simulink model "ME598A_Final_Project_R6"  (R2025b)
settings: Solver=ode23t  StartTime=0.0  StopTime=inf  RelTol=1e-3
InitFcn:
  | RPInit
model workspace (MAT data in the model file):
  mapForSim.obsMap = [0 0 0 0 0 0 0 0 0 0 0 0 ... (4194304 elements, 2048x2048)]
  mapForSim.scaleFactor = 409.6
  mapForSim.simMap = robotics.BinaryOccupancyGrid
  mapForSim.simMap.Grid = [1 1 1 1 1 1 1 1 1 1 1 1 ... (4194304 elements, 2048x2048)]
  mapForSim.simMap.SharedProperties = matlabshared.autonomous.internal.SharedMapProperties
  mapForSim.simMap.SharedProperties.Resolution = 409.6
  mapForSim.simMap.SharedProperties.GridSize = [2048 2048]
  mapForSim.simMap.SharedProperties.XLocalLimits = [0 5]
  mapForSim.simMap.SharedProperties.YLocalLimits = [0 5]
  mapForSim.simMap.SharedProperties.XWorldLimits = [0 5]
  mapForSim.simMap.SharedProperties.YWorldLimits = [0 5]
  mapForSim.simMap.SharedProperties.Width = 5
  mapForSim.simMap.SharedProperties.Height = 5
  mapForSim.simMap.SharedProperties.LocalOriginInWorldInternal = [0 0]
  mapForSim.simMap.LayerName = 'binaryLayer'
  mapForSim.simMap.DataType = 'logical'
  mapForSim.simMap.Buffer = matlabshared.autonomous.internal.CircularBuffer
  mapForSim.simMap.Buffer.ConstVal = 0
  mapForSim.simMap.Buffer.DataType = 'logical'
  mapForSim.simMap.Buffer.Index = matlabshared.autonomous.internal.CircularBufferIndex
  mapForSim.simMap.Buffer.Index.Head = [1 1]
  mapForSim.simMap.Buffer.Index.Size = [2048 2048]
  mapForSim.simMap.Buffer.Index.NewRegions = [0 0 0 0]
  mapForSim.simMap.Buffer.Index.DropEntireMap = 0
  mapForSim.simMap.Buffer.Index.DropTwoRegions = [0 0]
  mapForSim.simMap.Buffer.Buffer = [1 1 1 1 1 1 1 1 1 1 1 1 ... (4194304 elements, 2048x2048)]
  mapForSim.simMap.Buffer.BufferSize = [2048 2048 1]
  mapForSim.simMap.DefaultValueInternal = 0
  mapForSim.simMap.DataSize = [2048 2048]
  occGrid = robotics.BinaryOccupancyGrid
  occGrid.Grid = [1 1 1 1 1 1 1 1 1 1 1 1 ... (4194304 elements, 2048x2048)]
  occGrid.SharedProperties = matlabshared.autonomous.internal.SharedMapProperties
  occGrid.SharedProperties.Resolution = 409.6
  occGrid.SharedProperties.GridSize = [2048 2048]
  occGrid.SharedProperties.XLocalLimits = [0 5]
  occGrid.SharedProperties.YLocalLimits = [0 5]
  occGrid.SharedProperties.XWorldLimits = [0 5]
  occGrid.SharedProperties.YWorldLimits = [0 5]
  occGrid.SharedProperties.Width = 5
  occGrid.SharedProperties.Height = 5
  occGrid.SharedProperties.LocalOriginInWorldInternal = [0 0]
  occGrid.LayerName = 'binaryLayer'
  occGrid.DataType = 'logical'
  occGrid.Buffer = matlabshared.autonomous.internal.CircularBuffer
  occGrid.Buffer.ConstVal = 0
  occGrid.Buffer.DataType = 'logical'
  occGrid.Buffer.Index = matlabshared.autonomous.internal.CircularBufferIndex
  occGrid.Buffer.Index.Head = [1 1]
  occGrid.Buffer.Index.Size = [2048 2048]
  occGrid.Buffer.Index.NewRegions = [0 0 0 0]
  occGrid.Buffer.Index.DropEntireMap = 0
  occGrid.Buffer.Index.DropTwoRegions = [0 0]
  occGrid.Buffer.Buffer = [1 1 1 1 1 1 1 1 1 1 1 1 ... (4194304 elements, 2048x2048)]
  occGrid.Buffer.BufferSize = [2048 2048 1]
  occGrid.DefaultValueInternal = 0
  occGrid.DataSize = [2048 2048]
undefined symbols (not defined in the file): Base, FloorSurface, PlowSurface, Ref, RobotSurface, Side1, Side2, X, Y, Z
libraries: sm_lib x27, nesl_utility x11, RP_Simulator_Components x7, ME598_ProjectLibrary x3, RoboticsPlayground x2
(part 1 of 2)
settings Model: PacingRate=1000  Creator=josea  LastModifiedBy=beaut
settings SolverCC: AlgebraicLoopSolver=TrustRegion
settings DataIOCC: ReturnWorkspaceOutputs=off
settings DebuggingCC: UnconnectedInputMsg=warning  UnconnectedOutputMsg=warning  ArithmeticOperatorsInVariantConditions=warning
settings ModelReferenceCC: EnableRefExpFcnMdlSchedulingChecks=on
settings SFSimCC: SimUseLocalCustomCode=off  CustomCodeUndefinedFunction=UseInterfaceOnly
settings RTWCC: RTWUseLocalCustomCode=off  GPUComputeCapability=3.5  DLArmComputeVersion=19.05
settings DiagnosticsConfigSet: SimMechanicsRigidlyBoundBlock=none
settings ExplorerConfigSet: InternalSimMechanicsExplorerSettings="<ExplorerConfiguration><canonicalview>default</canonicalview><TilePanel><TileInfo><Tiles Columns=\"2\" Count=\"3\" Height=\"704\" Rows=\"2\" Width=\"1079\"><Row Weight=\"0.4995\"/><Row Weight=\"0.5005\"/><Column Weight=\"0.4996\"/><Column Weight=\"0.5004\"/><Tile Height=\"1\" Width=\"2\" X=\"0\" Y=\"0\"/><Tile Height=\"1\" Width=\"1\" X=\"0\" Y=\"1\"/><Tile Height=\"1\" Width=\"1\" X=\"1\" Y=\"1\"/></Tiles></TileInfo><SceneInfo><SceneViewer><IsThisViewStd><IsStandardView>off</IsStandardView><StandardViewName>Front</StandardViewName></IsThisViewStd><BGColor><R>0.60000002384185791</R><G>0.60000002384185791</G><B>0.60000002384185791</B><A>1</A></BGColor><Camera><DoPerspective>off</DoPerspective><Position><X>-0.86116534267326283</X><Y>0.23588412890430099</Y><Z>21.59798</Z></Position><Center><X>-0.86116534267326283</X><Y>0.23588412890430099</Y><Z>0.12587000000000001</Z></Center><Up><X>0</X><Y>1</Y><Z>0</Z></Up><XLim>3.0477928446452562</XLim><YLim>3.0477928446452562</YLim><ViewLimDist>0.01</ViewLimDist></Camera></SceneViewer><SceneViewer><IsThisViewStd><IsStandardView>off</IsStandardView><StandardViewName>Front</StandardViewName></IsThisViewStd><BGColor><R>0.60000002384185791</R><G>0.60000002384185791</G><B>0.60000002384185791</B><A>1</A></BGColor><Camera><DoPerspective>on</DoPerspective><Position><X>-0.46788000000000002</X><Y>0.21970000000000001</Y><Z>0.45108999999999999</Z></Position><Center><X>0.46222000000000002</X><Y>0.085760000000000003</Y><Z>0.10907</Z></Center><Up><X>0.33852730030170697</X><Y>-0.048749611226549958</Y><Z>0.9396928978957424</Z></Up><XLim>0.46630765815499858</XLim><YLim>0.46630765815499858</YLim><ViewLimDist>0.01</ViewLimDist></Camera></SceneViewer><SceneViewer><IsThisViewStd><IsStandardView>off</IsStandardView><StandardViewName>Front</StandardViewName></IsThisViewStd><BGColor><R>0.60000002384185791</R><G>0.60000002384185791</G><B>0.60000002384185791</B><A>1</A></BGColor><Camera><DoPerspective>off</DoPerspective><Position><X>0</X><Y>0</Y><Z>21.59798</Z></Position><Center><X>0</X><Y>0</Y><Z>0.12587000000000001</Z></Center><Up><X>0</X><Y>1</Y><Z>0</Z></Up><XLim>2.5955999995395542</XLim><YLim>2.5955999995395542</YLim><ViewLimDist>0.01</ViewLimDist></Camera></SceneViewer></SceneInfo></TilePanel><MechEditorPanel><GfxPanelCameraMap><MapElement CameraMLId=\"Camera1\" GfxPanelIndex=\"1\"/></GfxPanelCameraMap><Cameras><Camera><Id>Camera1</Id><Value><Name>RobotView</Name><NativeCamera><PositionTrackingFeature>Object_Environment_ME_598.Plow_Tank_Robot.Body.RobotCamera.F</PositionTrackingFeature><CenterTrackingFeature>Object_Environment_ME_598.Plow_Tank_Robot.Body.RobotCamera.F</CenterTrackingFeature><UpVectorTrackingFeature>Object_Environment_ME_598.Plow_Tank_Robot.Body.RobotCamera.F</UpVectorTrackingFeature><CenterTrackingOrigin>off</CenterTrackingOrigin><CenterTrackingDirection>+X</CenterTrackingDirection><UpVectorTrackingDirection>+Z</UpVectorTrackingDirection></NativeCamera></Value></Camera></Cameras><VideoCreator><IncludeTiles>Selected</IncludeTiles><IncludeTime>on</IncludeTime><IncludeWorldFrame>off</IncludeWorldFrame><PlaybackSpeedRatio>1</PlaybackSpeedRatio><FrameRate>30</FrameRate><FrameSize>auto</FrameSize><VideoFormat>MotionJPEGAVI</VideoFormat></VideoCreator></MechEditorPanel><PlaybackSettings><PlaybackSpeedFactor>4</PlaybackSpeedFactor></PlaybackSettings></ExplorerConfiguration>"

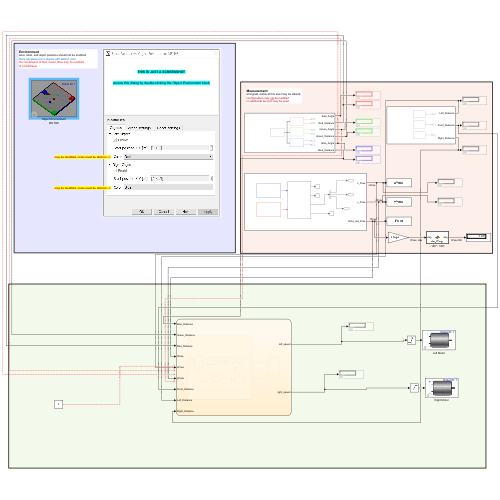
[thumbnail: Simulink's stored preview of the top-level diagram]
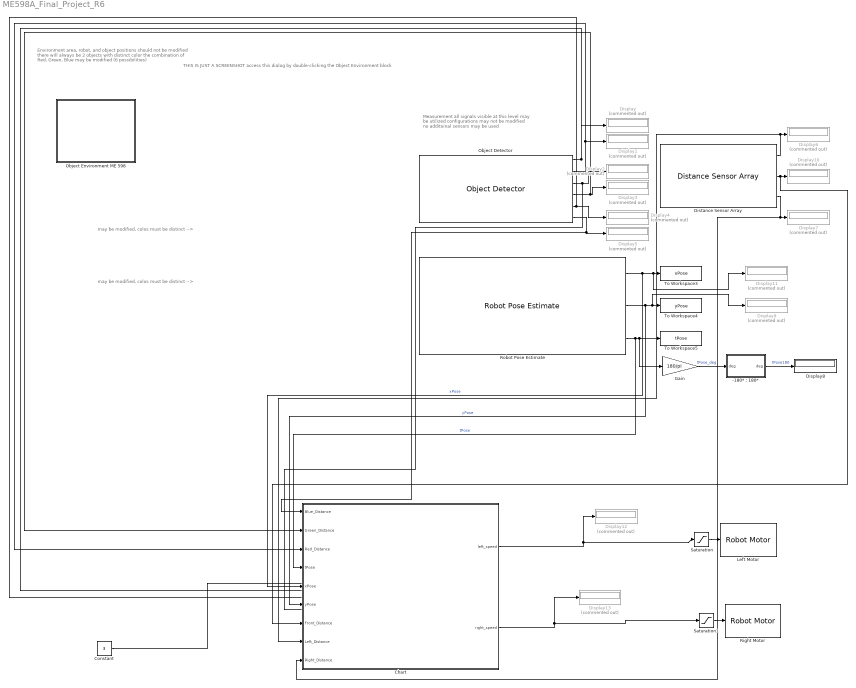
== system ME598A_Final_Project_R6 ==
  note: Environment
      | area, robot, and object positions should not be modified
      | there will always be 2 objects with distinct color
      | the combination of Red, Green, Blue may be modified
      | (6 possibilities)
  note: Measurement
      | all signals visible at this level may be utilized configurations may not be modified
      | no additoinal sensors may be used
  note: may be modified, colos must be distinct -->
  note: THIS IS JUST A SCREENSHOT
      |
      | access this dialog by double-clicking the Object Environment block
  note: may be modified, colos must be distinct -->
  "-180* : 180*" : MATLAB Function  TreatAsAtomicUnit=on
  Chart : Stateflow chart  TreatAsAtomicUnit=on
  Constant : Constant  Value=3
  Display{,1..7,9..13} (13 alike) : Display  Commented=on
  Display8 : Display
  Distance Sensor Array : ME598_ProjectLibrary/Distance Sensor Array
  Gain : Gain  Gain=180/pi
  Left Motor : RoboticsPlayground/Basic Sensors and Actuators/Robot Motor  robotId=1  motorChoice=1
      settings: SourceProductName=Robotics Playground
  Object Detector : ME598_ProjectLibrary/Object Detector
  Object Environment ME 598 : Subsystem  mask(RP Object Environment){obj1=on, objPose1=[0 1.5], objColor1=Green, obj2=off, objPose2=[0 0], objColor2=Green, obj3=on, objPose3=[0 -1.5], objColor3=Red, obj4=off, objPose4=[-0.61298      2.9263], objColor4=Red, obj5=off, objPose5=[-0.61298      2.9263], objColor5=Red, arenaLength=5, arenaWidth=5, robotId=1, wheelBase=0.5, wheelRadius=0.1, robotColor=[0.5 0 0], startPose=[-1.5 -1.5]}
      mask prompts: obj1 "Enabled"; objPose1 "Initial position X Y [m]"; objColor1 "Color"; obj2 "Enabled"; objPose2 "Initial position X Y [m]"; objColor2 "Color"; obj3 "Enabled"; objPose3 "Initial position X Y [m]"; objColor3 "Color"; obj4 "Enabled"; objPose4 "Initial position X Y [m]"; objColor4 "Color"; obj5 "Enabled"; objPose5 "Initial position X Y [m]"; objColor5 "Color"; arenaLength "Length [m]"; arenaWidth "Width [m]"; robotId "Robot ID"; wheelBase "Distance between wheels [m]"; wheelRadius "Wheel radius [m]"; robotColor "Color [R G B]"; startPose "Initial Position X Y [m]"
      mask help:
      | This block has been customized and tested with MATLAB R2025b and Robotics Playground v23.1.1.0
      | for Stevens Institute of Technology course ME 598, Spring 2026.
      |
      | It contains a virtual environment for a single robot to interact with walls and moveable objects. For your course project, only the sensors and actuators provided in the file ** Project_start.slx ** may be used for sensing and to actuate the robot.
      |
      | Motor mapping for the robot is as follows:
      |
      | Motor 1 -> Left wheel motor **torque**
      | Motor 2 -> Right wheel motor **torque**
      settings: CopyFcn=|
      | set_param(gcs,'InitFcn','RPInit');
      | set_param(gcs,'Solver','ode23t');
      | set_param(gcs, 'EnablePacing', 'on')
      | set_param(gcs, 'PacingRate', 1)
      mask Help: web('object_arena.htm')
      mask Callback obj1: setObjects(gcb)
      mask Callback objPose1: setObjects(gcb)
      mask TypeOptions objColor1: Red | Green | Blue
      mask Callback objColor1: setObjects(gcb)
      mask Callback obj2: setObjects(gcb)
      mask Callback objPose2: setObjects(gcb)
      mask TypeOptions objColor2: Red | Green | Blue
      mask Callback objColor2: setObjects(gcb)
      mask Callback obj3: setObjects(gcb)
      mask Callback objPose3: setObjects(gcb)
      mask TypeOptions objColor3: Red | Green | Blue
      mask Callback objColor3: setObjects(gcb)
      mask Callback obj4: setObjects(gcb)
      mask Callback objPose4: setObjects(gcb)
      mask TypeOptions objColor4: Red | Green | Blue
      mask Callback objColor4: setObjects(gcb)
      mask Callback obj5: setObjects(gcb)
      mask Callback objPose5: setObjects(gcb)
      mask TypeOptions objColor5: Red | Green | Blue
      mask Callback objColor5: setObjects(gcb)
      mask DialogControl objT Prompt: Object settings
      mask DialogControl objc1 Prompt: Left Object
      mask DialogControl objc2 Prompt: Center Object
      mask DialogControl objc3 Prompt: Right Object
      mask DialogControl objc4 Prompt: Object 4
      mask DialogControl objc5 Prompt: Object 5
      mask DialogControl Container6 Prompt: Arena settings
      mask DialogControl Container4 Prompt: Robot settings
      mask Display:
      | color('white');
      | plot([100,100,100,100]*1,[100,100,100,100]*1);
      | plot([100,100,100,100]*0,[100,100,100,100]*0);
      | image('ObjectEnv.PNG')
      | color('blue');
      | id=eval(get_param(gcb,'robotId'));
      | text(99, 92, ['Robot ID: ' num2str(id)], 'horizontalAlignment', 'right');
  Right Motor : RoboticsPlayground/Basic Sensors and Actuators/Robot Motor  robotId=1  motorChoice=2
      settings: SourceProductName=Robotics Playground
  Robot Pose Estimate : ME598_ProjectLibrary/Robot Pose Estimate
  Saturation : Saturate  UpperLimit=127  LowerLimit=-127
  Saturation1 : Saturate  UpperLimit=127  LowerLimit=-127
  To Workspace3 : ToWorkspace  VariableName=xPose  SampleTime=-1
  To Workspace4 : ToWorkspace  VariableName=yPose  SampleTime=-1
  To Workspace5 : ToWorkspace  VariableName=tPose  SampleTime=-1
  wires:
  Object Detector/1 -> Display/1
  Object Detector/2 -> Chart/3(Red_Distance), Display1/1
  Object Detector/4 -> Chart/2(Green_Distance), Display3/1
  Object Detector/3 -> Display2/1
  Distance Sensor Array/1 -> Chart/8(Left_Distance), Display6/1
  Distance Sensor Array/3 -> Chart/9(Right_Distance), Display7/1
  Robot Pose Estimate/3 -> Chart/4(tPose), Gain/1, To Workspace5/1  "tPose"
  Gain/1 -> "-180* : 180*"/1("deg ")  "tPose_deg"
  Robot Pose Estimate/1 -> Chart/5(xPose), Display11/1, To Workspace3/1  "xPose"
  Robot Pose Estimate/2 -> Chart/6(yPose), Display9/1, To Workspace4/1  "yPose"
  Saturation/1 -> Left Motor/1
  Distance Sensor Array/2 -> Chart/7(Front_Distance), Display10/1
  "-180* : 180*"/1(deg) -> Display8/1  "tPose180"
  Object Detector/5 -> Display4/1
  Object Detector/6 -> Chart/1(Blue_Distance), Display5/1
  Saturation1/1 -> Right Motor/1
  Chart/1(left_speed) -> Display12/1, Saturation/1
  Chart/2(right_speed) -> Display13/1, Saturation1/1
  Constant/1 -> ?

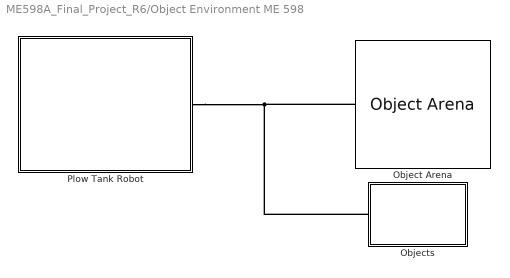
== system ME598A_Final_Project_R6/Object Environment ME 598 ==
  Object Arena : RP_Simulator_Components/Object Arena  length=arenaLength  width=arenaWidth  robotRadius=wheelBase/2
  Objects : Subsystem
  Plow Tank Robot : Subsystem  AncestorBlock=RoboticsPlayground/Environments/Object Environment/Plow Tank Robot  mask(RP Contact Tank Robot){robotId=robotId, wheelRadius=wheelRadius, wheelBase=wheelBase, wheelThickness=0.025, chassisThickness=0.05, startPose=startPose, choice=off, sensorTs=0.05, wheelMass=0.2, chassisMass=0.5, maxWheelTorque=1, floorSize=[arenaLength arenaWidth], wheelColor=[0.25 0.25 0.25], chassisColor=robotColor}
      mask prompts: robotId "Robot ID"; wheelRadius "Wheel Radius [m]"; wheelBase "Wheelbase [m]"; wheelThickness "Wheel Thickness [m]"; chassisThickness "Chassis Thickness [m]"; startPose "Start Position [m]"; choice "Reverse Start Position"; sensorTs "Sensor sample time [s]"; wheelMass "Wheel Mass [kg]"; chassisMass "Chassis Mass [kg]"; maxWheelTorque "Maximum wheel torque [N*m]"; floorSize "Floor Dimensions [m]"; wheelColor "Wheel Color"; chassisColor "Chassis Color"
      mask help:
      | This robot implements contact between the robot wheels and the floor of an arena. The stck-slip friction implemented using contact force libraries makes the robot behavior more realistic. The inputs to the robot are now motor torque, which is set using the Robotics Playground Motor blocks. The motor mappings are as follows:
      |
      | Motor 1 -> Left wheel motor torque
      | Motor 2 -> Right wheel motor torque
      mask init:
      | ID=num2str(eval(get_param(gcb,'robotId')));
      | block=gcb;
      | 
      | set_param([block '/motor1t'],'GotoTag',['R' ID 'motor1t']);
      | set_param([block '/motor2t'],'GotoTag',['R' ID 'motor2t']);
      | set_param([block '/motor1q'],'GotoTag',['R' ID 'motor1q']);
      | set_param([block '/motor1w'],'GotoTag',['R' ID 'motor1w']);
      | set_param([block '/motor2q'],'GotoTag',['R' ID 'motor2q']);
      | set_param([block '/motor2w'],'GotoTag',['R' ID 'motor2w']);
      | set_param([block '/xPose'],'GotoTag',['R' ID 'xPose']);
      | set_param([block '/yPose'],'GotoTag',['R' ID 'yPose']);
      | set_param([block '/tPose'],'GotoTag',['R' ID 'tPose']);
      | set_param([block '/tRate'],'GotoTag',['R' ID 'tRate']);
      | set_param([block '/tAngle'],'GotoTag',['R' ID 'tAngle']);
      | 
      | % Add sensor visuals
      | 
      | addSensors(block,eval(ID));
      mask DialogControl KinContainer Prompt: Kinematics
      mask DialogControl DynamicsContainer Prompt: Dynamics
      mask DialogControl AppearanceContainer Prompt: Appearance
      mask Display:
      | image('plowRobot.PNG')
      | port_label('Rconn',1,'RP-Bus')
  connections:
  Object Arena/LConn1 -- Plow Tank Robot/RConn1 -- Objects/LConn1

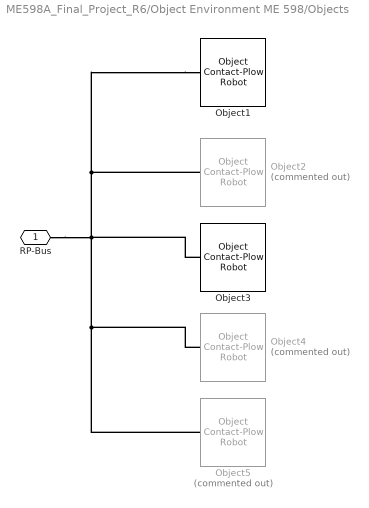
== system ME598A_Final_Project_R6/Object Environment ME 598/Objects ==
  Object1 : RP_Simulator_Components/Object Contact-Plow Robot  objectId=1  Pose=[0 1.5]  objRadius=0.15  robotRadius=0.25  height=0.2  color=[0 0.8 0]  length=arenaLength  width=arenaWidth
  Object2 : RP_Simulator_Components/Object Contact-Plow Robot  Commented=on  objectId=2  Pose=[0 0]  objRadius=0.15  robotRadius=0.25  height=0.2  color=[0 0.8 0]  length=arenaLength  width=arenaWidth
  Object3 : RP_Simulator_Components/Object Contact-Plow Robot  objectId=3  Pose=[0 -1.5]  objRadius=0.15  robotRadius=0.25  height=0.2  color=[0.8 0 0]  length=arenaLength  width=arenaWidth
  Object4 : RP_Simulator_Components/Object Contact-Plow Robot  Commented=on  objectId=4  Pose="[-0.61298      2.9263]"  objRadius=0.15  robotRadius=0.25  height=0.2  color=[0.8 0 0]  length=arenaLength  width=arenaWidth
  Object5 : RP_Simulator_Components/Object Contact-Plow Robot  Commented=on  objectId=5  Pose="[-0.61298      2.9263]"  objRadius=0.15  robotRadius=0.25  height=0.2  color=[0.8 0 0]  length=arenaLength  width=arenaWidth
  RP-Bus : PMIOPort  Side=Left
  connections:
  Object1/LConn1 -- Object3/LConn1 -- Object5/LConn1 -- Object4/LConn1 -- RP-Bus/RConn1 -- Object2/LConn1

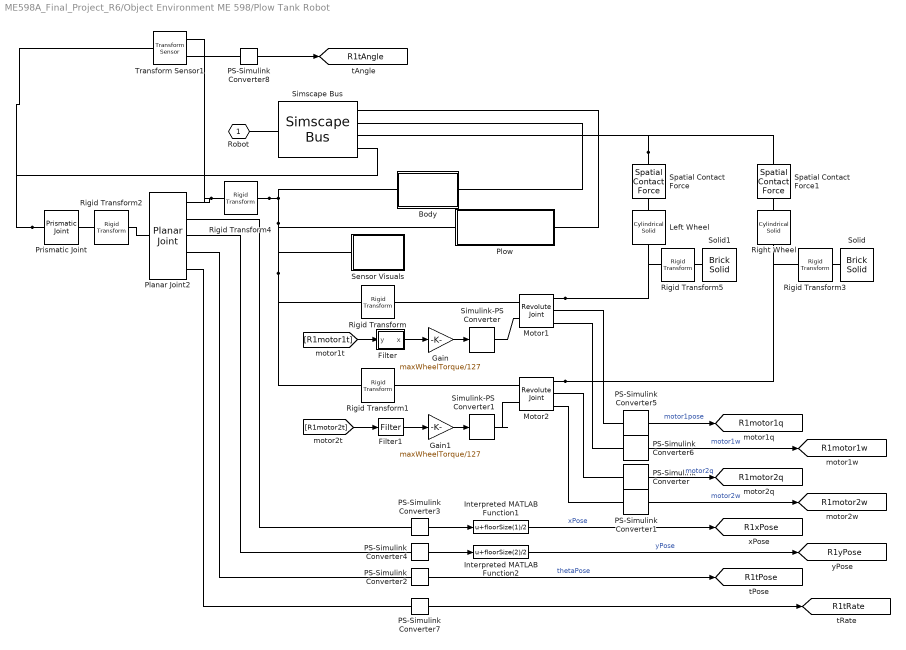
== system ME598A_Final_Project_R6/Object Environment ME 598/Plow Tank Robot ==
  Body : Subsystem
  Filter : Subsystem
  Filter1 : RP_Simulator_Components/Contact Tank Robot/Filter  SystemSampleTime=-1  VariantActivationTime=update diagram  EmptyChoice=off  PassThrough=off  PassThroughVariantControl=(default)  EmptyChoiceVariantControl=(default)  AllowFlexibleInterface=on  Latency=0  AutoFrameSizeCalculation=off
  Gain : Gain  Gain=maxWheelTorque/127
  Gain1 : Gain  Gain=maxWheelTorque/127
  Interpreted MATLAB Function1 : MATLABFcn  MATLABFcn=u+floorSize(1)/2
  Interpreted MATLAB Function2 : MATLABFcn  MATLABFcn=u+floorSize(2)/2
  Left Wheel : sm_lib/Body Elements/Cylindrical Solid  CylinderRadius=wheelRadius  CylinderRadiusUnits=m  CylinderLength=wheelThickness  CylinderLengthUnits=m  ExportEntireGeometry=on  InertiaType=CalculateFromGeometry  BasedOnType=Mass  Density=1000  DensityUnits=kg/m^3  Mass=wheelMass  MassUnits=kg  CenterOfMass=[0 0 0]  CenterOfMassUnits=m  MomentsOfInertia=[1 1 1]  MomentsOfInertiaUnits=kg*m^2  ProductsOfInertia=[1 1 1]  ProductsOfInertiaUnits=kg*m^2  GraphicType=FromGeometry  MarkerShape=Sphere  MarkerSize=10  GraphicVisPropType=SimpleVisualProperties  GraphicDiffuseColor=wheelColor  GraphicOpacity=1.0  GraphicSpecularColor=[0.5 0.5 0.5 1.0]  GraphicAmbientColor=[0.15 0.15 0.15 1.0]  GraphicEmissiveColor=[0.0 0.0 0.0 1.0]  GraphicShininess=75  DoExposeReferenceFrame=on  SerializedFrames=<Frames/>
  Motor1 : sm_lib/Joints/Revolute Joint  JointMode=Normal  CompositeWrenchDir=FollowerOnBase  CompositeWrenchFrame=BaseFrame  SenseConstraintForce=off  SenseConstraintTorque=off  SenseTotalForce=off  SenseTotalTorque=off  PositionTargetSpecify=off  PositionTargetPriority=High  PositionTargetValue=0  PositionTargetValueUnits=deg  VelocityTargetSpecify=off  VelocityTargetPriority=High  VelocityTargetValue=0  VelocityTargetValueUnits=deg/s  EquilibriumPosition=0  EquilibriumPositionUnits=deg  SpringStiffness=0  SpringStiffnessUnits=N*m/deg  DampingCoefficient=0.004  DampingCoefficientUnits=N*m/(deg/s)  LowerLimitSpecify=off  LowerLimitBound=-90  LowerLimitBoundUnits=deg  LowerLimitStiffness=1e4  LowerLimitStiffnessUnits=N*m/deg  LowerLimitDamping=10  LowerLimitDampingUnits=N*m/(deg/s)  LowerLimitTransitionRegionWidth=0.1  LowerLimitTransitionRegionWidthUnits=deg  UpperLimitSpecify=off  UpperLimitBound=90  UpperLimitBoundUnits=deg  UpperLimitStiffness=1e4  UpperLimitStiffnessUnits=N*m/deg  UpperLimitDamping=10  UpperLimitDampingUnits=N*m/(deg/s)  UpperLimitTransitionRegionWidth=0.1  UpperLimitTransitionRegionWidthUnits=deg  TorqueActuationMode=InputTorque  MotionActuationMode=ComputedMotion  SensePosition=on  SenseVelocity=on  SenseAcceleration=off  SenseTorqueForce=off  SenseLowerLimitTorqueForce=off  SenseUpperLimitTorqueForce=off
  Motor2 : sm_lib/Joints/Revolute Joint  JointMode=Normal  CompositeWrenchDir=FollowerOnBase  CompositeWrenchFrame=BaseFrame  SenseConstraintForce=off  SenseConstraintTorque=off  SenseTotalForce=off  SenseTotalTorque=off  PositionTargetSpecify=off  PositionTargetPriority=High  PositionTargetValue=0  PositionTargetValueUnits=deg  VelocityTargetSpecify=off  VelocityTargetPriority=High  VelocityTargetValue=0  VelocityTargetValueUnits=deg/s  EquilibriumPosition=0  EquilibriumPositionUnits=deg  SpringStiffness=0  SpringStiffnessUnits=N*m/deg  DampingCoefficient=0.004  DampingCoefficientUnits=N*m/(deg/s)  LowerLimitSpecify=off  LowerLimitBound=-90  LowerLimitBoundUnits=deg  LowerLimitStiffness=1e4  LowerLimitStiffnessUnits=N*m/deg  LowerLimitDamping=10  LowerLimitDampingUnits=N*m/(deg/s)  LowerLimitTransitionRegionWidth=0.1  LowerLimitTransitionRegionWidthUnits=deg  UpperLimitSpecify=off  UpperLimitBound=90  UpperLimitBoundUnits=deg  UpperLimitStiffness=1e4  UpperLimitStiffnessUnits=N*m/deg  UpperLimitDamping=10  UpperLimitDampingUnits=N*m/(deg/s)  UpperLimitTransitionRegionWidth=0.1  UpperLimitTransitionRegionWidthUnits=deg  TorqueActuationMode=InputTorque  MotionActuationMode=ComputedMotion  SensePosition=on  SenseVelocity=on  SenseAcceleration=off  SenseTorqueForce=off  SenseLowerLimitTorqueForce=off  SenseUpperLimitTorqueForce=off
  PS-Simulink Converter{,1,3..6} (6 alike) : nesl_utility/PS-Simulink Converter  PhysicalDomain=network_engine_domain  SubClassName=ps_output  LeftPortType=input  RightPortType=output  PseudoPeriodic=off  Frequencies=[]  VectorFormat=1-D array  Unit=1  AffineConversion=off
  PS-Simulink Converter2 : nesl_utility/PS-Simulink Converter  PhysicalDomain=network_engine_domain  SubClassName=ps_output  LeftPortType=input  RightPortType=output  PseudoPeriodic=off  Frequencies=[]  VectorFormat=1-D array  Unit=rad  AffineConversion=off
  PS-Simulink Converter7 : nesl_utility/PS-Simulink Converter  PhysicalDomain=network_engine_domain  SubClassName=ps_output  LeftPortType=input  RightPortType=output  PseudoPeriodic=off  Frequencies=[]  VectorFormat=1-D array  Unit=deg/s  AffineConversion=off
  PS-Simulink Converter8 : nesl_utility/PS-Simulink Converter  PhysicalDomain=network_engine_domain  SubClassName=ps_output  LeftPortType=input  RightPortType=output  PseudoPeriodic=off  Frequencies=[]  VectorFormat=1-D array  Unit=deg  AffineConversion=off
  Planar Joint2 : sm_lib/Joints/Planar Joint  JointMode=Normal  CompositeWrenchDir=FollowerOnBase  CompositeWrenchFrame=BaseFrame  SenseConstraintForce=off  SenseConstraintTorque=off  SenseTotalForce=off  SenseTotalTorque=off  PxPositionTargetSpecify=on  PxPositionTargetPriority=High  PxPositionTargetValue=startPose(1)  PxPositionTargetValueUnits=m  PxVelocityTargetSpecify=off  PxVelocityTargetPriority=High  PxVelocityTargetValue=0  PxVelocityTargetValueUnits=m/s  PxEquilibriumPosition=0  PxEquilibriumPositionUnits=m  PxSpringStiffness=0  PxSpringStiffnessUnits=N/m  PxDampingCoefficient=5  PxDampingCoefficientUnits=N/(m/s)  PxLowerLimitSpecify=off  PxLowerLimitBound=-1  PxLowerLimitBoundUnits=m  PxLowerLimitStiffness=1e6  PxLowerLimitStiffnessUnits=N/m  PxLowerLimitDamping=1e3  PxLowerLimitDampingUnits=N/(m/s)  PxLowerLimitTransitionRegionWidth=1e-4  PxLowerLimitTransitionRegionWidthUnits=m  PxUpperLimitSpecify=off  PxUpperLimitBound=1  PxUpperLimitBoundUnits=m  PxUpperLimitStiffness=1e6  PxUpperLimitStiffnessUnits=N/m  PxUpperLimitDamping=1e3  PxUpperLimitDampingUnits=N/(m/s)  PxUpperLimitTransitionRegionWidth=1e-4  PxUpperLimitTransitionRegionWidthUnits=m  PxTorqueActuationMode=NoTorque  PxMotionActuationMode=ComputedMotion  PxSensePosition=on  PxSenseVelocity=off  PxSenseAcceleration=off  PxSenseTorqueForce=off  PxSenseLowerLimitTorqueForce=off  PxSenseUpperLimitTorqueForce=off  PyPositionTargetSpecify=on  PyPositionTargetPriority=High  PyPositionTargetValue=startPose(2)  PyPositionTargetValueUnits=m  PyVelocityTargetSpecify=off  PyVelocityTargetPriority=High  PyVelocityTargetValue=0  PyVelocityTargetValueUnits=m/s  PyEquilibriumPosition=0  PyEquilibriumPositionUnits=m  PySpringStiffness=0  PySpringStiffnessUnits=N/m  PyDampingCoefficient=5  PyDampingCoefficientUnits=N/(m/s)  PyLowerLimitSpecify=off  PyLowerLimitBound=-1  PyLowerLimitBoundUnits=m  PyLowerLimitStiffness=1e6  PyLowerLimitStiffnessUnits=N/m  PyLowerLimitDamping=1e3  PyLowerLimitDampingUnits=N/(m/s)  PyLowerLimitTransitionRegionWidth=1e-4  PyLowerLimitTransitionRegionWidthUnits=m  PyUpperLimitSpecify=off  PyUpperLimitBound=1  PyUpperLimitBoundUnits=m  PyUpperLimitStiffness=1e6  PyUpperLimitStiffnessUnits=N/m  PyUpperLimitDamping=1e3  PyUpperLimitDampingUnits=N/(m/s)  PyUpperLimitTransitionRegionWidth=1e-4  PyUpperLimitTransitionRegionWidthUnits=m  PyTorqueActuationMode=NoTorque  PyMotionActuationMode=ComputedMotion  PySensePosition=on  PySenseVelocity=off  PySenseAcceleration=off  PySenseTorqueForce=off  PySenseLowerLimitTorqueForce=off  PySenseUpperLimitTorqueForce=off  RzPositionTargetSpecify=off  RzPositionTargetPriority=High  RzPositionTargetValue=0  RzPositionTargetValueUnits=deg  RzVelocityTargetSpecify=off  RzVelocityTargetPriority=High  RzVelocityTargetValue=0  RzVelocityTargetValueUnits=deg/s  RzEquilibriumPosition=0  RzEquilibriumPositionUnits=deg  RzSpringStiffness=0  RzSpringStiffnessUnits=N*m/deg  RzDampingCoefficient=2/45  RzDampingCoefficientUnits=N*m/(deg/s)  RzLowerLimitSpecify=off  RzLowerLimitBound=-90  RzLowerLimitBoundUnits=deg  RzLowerLimitStiffness=1e4  RzLowerLimitStiffnessUnits=N*m/deg  RzLowerLimitDamping=10  RzLowerLimitDampingUnits=N*m/(deg/s)  RzLowerLimitTransitionRegionWidth=0.1  RzLowerLimitTransitionRegionWidthUnits=deg  RzUpperLimitSpecify=off  RzUpperLimitBound=90  RzUpperLimitBoundUnits=deg  RzUpperLimitStiffness=1e4  RzUpperLimitStiffnessUnits=N*m/deg  RzUpperLimitDamping=10  RzUpperLimitDampingUnits=N*m/(deg/s)  RzUpperLimitTransitionRegionWidth=0.1  RzUpperLimitTransitionRegionWidthUnits=deg  RzTorqueActuationMode=NoTorque  RzMotionActuationMode=ComputedMotion  RzSensePosition=on  RzSenseVelocity=on  RzSenseAcceleration=off  RzSenseTorqueForce=off  RzSenseLowerLimitTorqueForce=off  RzSenseUpperLimitTorqueForce=off
  Plow : Subsystem
  Prismatic Joint : sm_lib/Joints/Prismatic Joint  JointMode=Normal  CompositeWrenchDir=FollowerOnBase  CompositeWrenchFrame=BaseFrame  SenseConstraintForce=off  SenseConstraintTorque=off  SenseTotalForce=off  SenseTotalTorque=off  PositionTargetSpecify=on  PositionTargetPriority=High  PositionTargetValue=0.02  PositionTargetValueUnits=m  VelocityTargetSpecify=off  VelocityTargetPriority=High  VelocityTargetValue=0  VelocityTargetValueUnits=m/s  EquilibriumPosition=0  EquilibriumPositionUnits=m  SpringStiffness=0  SpringStiffnessUnits=N/m  DampingCoefficient=0  DampingCoefficientUnits=N/(m/s)  LowerLimitSpecify=off  LowerLimitBound=-1  LowerLimitBoundUnits=m  LowerLimitStiffness=1e6  LowerLimitStiffnessUnits=N/m  LowerLimitDamping=1e3  LowerLimitDampingUnits=N/(m/s)  LowerLimitTransitionRegionWidth=1e-4  LowerLimitTransitionRegionWidthUnits=m  UpperLimitSpecify=off  UpperLimitBound=1  UpperLimitBoundUnits=m  UpperLimitStiffness=1e6  UpperLimitStiffnessUnits=N/m  UpperLimitDamping=1e3  UpperLimitDampingUnits=N/(m/s)  UpperLimitTransitionRegionWidth=1e-4  UpperLimitTransitionRegionWidthUnits=m  TorqueActuationMode=NoTorque  MotionActuationMode=ComputedMotion  SensePosition=off  SenseVelocity=off  SenseAcceleration=off  SenseTorqueForce=off  SenseLowerLimitTorqueForce=off  SenseUpperLimitTorqueForce=off
  Right Wheel : sm_lib/Body Elements/Cylindrical Solid  CylinderRadius=wheelRadius  CylinderRadiusUnits=m  CylinderLength=wheelThickness  CylinderLengthUnits=m  ExportEntireGeometry=on  InertiaType=CalculateFromGeometry  BasedOnType=Mass  Density=1000  DensityUnits=kg/m^3  Mass=wheelMass  MassUnits=kg  CenterOfMass=[0 0 0]  CenterOfMassUnits=m  MomentsOfInertia=[1 1 1]  MomentsOfInertiaUnits=kg*m^2  ProductsOfInertia=[1 1 1]  ProductsOfInertiaUnits=kg*m^2  GraphicType=FromGeometry  MarkerShape=Sphere  MarkerSize=10  GraphicVisPropType=SimpleVisualProperties  GraphicDiffuseColor=wheelColor  GraphicOpacity=1.0  GraphicSpecularColor=[0.5 0.5 0.5 1.0]  GraphicAmbientColor=[0.15 0.15 0.15 1.0]  GraphicEmissiveColor=[0.0 0.0 0.0 1.0]  GraphicShininess=75  DoExposeReferenceFrame=on  SerializedFrames=<Frames/>
  Rigid Transform : sm_lib/Frames and Transforms/Rigid Transform  RotationMethod=AlignedAxes  FollAlignAxisA=+Z  BaseAlignAxisA=+Y  FollAlignAxisB=+X  BaseAlignAxisB=+X  RotationStandardAxis=+Z  RotationAngle=0.0  RotationAngleUnits=deg  RotationArbitraryAxis=[0 0 1]  RotationSequenceAxes=FollowerAxes  RotationSequence=XYX  RotationSequenceAngles=[0 0 0]  RotationSequenceAnglesUnits=deg  RotationMatrix=[1 0 0; 0 1 0; 0 0 1]  Quaternion=[1 0 0 0]  TranslationMethod=StandardAxis  TranslationCartesianOffset=[0 0 0]  TranslationCartesianOffsetUnits=m  TranslationStandardAxis=+Y  TranslationStandardOffset=wheelBase/2  TranslationStandardOffsetUnits=m  TranslationROffset=0  TranslationROffsetUnits=m  TranslationThetaOffset=0  TranslationThetaOffsetUnits=deg  TranslationZOffset=0  TranslationZOffsetUnits=m
  Rigid Transform1 : sm_lib/Frames and Transforms/Rigid Transform  RotationMethod=AlignedAxes  FollAlignAxisA=+Z  BaseAlignAxisA=+Y  FollAlignAxisB=+X  BaseAlignAxisB=+X  RotationStandardAxis=+Z  RotationAngle=0.0  RotationAngleUnits=deg  RotationArbitraryAxis=[0 0 1]  RotationSequenceAxes=FollowerAxes  RotationSequence=XYX  RotationSequenceAngles=[0 0 0]  RotationSequenceAnglesUnits=deg  RotationMatrix=[1 0 0; 0 1 0; 0 0 1]  Quaternion=[1 0 0 0]  TranslationMethod=StandardAxis  TranslationCartesianOffset=[0 0 0]  TranslationCartesianOffsetUnits=m  TranslationStandardAxis=-Y  TranslationStandardOffset=wheelBase/2  TranslationStandardOffsetUnits=m  TranslationROffset=0  TranslationROffsetUnits=m  TranslationThetaOffset=0  TranslationThetaOffsetUnits=deg  TranslationZOffset=0  TranslationZOffsetUnits=m
  Rigid Transform2 : sm_lib/Frames and Transforms/Rigid Transform  RotationMethod=None  FollAlignAxisA=+Z  BaseAlignAxisA=+Y  FollAlignAxisB=+X  BaseAlignAxisB=+X  RotationStandardAxis=+Z  RotationAngle=0.0  RotationAngleUnits=deg  RotationArbitraryAxis=[0 0 1]  RotationSequenceAxes=FollowerAxes  RotationSequence=XYX  RotationSequenceAngles=[0 0 0]  RotationSequenceAnglesUnits=deg  RotationMatrix=[1 0 0; 0 1 0; 0 0 1]  Quaternion=[1 0 0 0]  TranslationMethod=StandardAxis  TranslationCartesianOffset=[0 0 0]  TranslationCartesianOffsetUnits=m  TranslationStandardAxis=+Z  TranslationStandardOffset=wheelRadius  TranslationStandardOffsetUnits=m  TranslationROffset=0  TranslationROffsetUnits=m  TranslationThetaOffset=0  TranslationThetaOffsetUnits=deg  TranslationZOffset=0  TranslationZOffsetUnits=m
  Rigid Transform3 : sm_lib/Frames and Transforms/Rigid Transform  RotationMethod=None  FollAlignAxisA=+X  BaseAlignAxisA=+Y  FollAlignAxisB=+Y  BaseAlignAxisB=+Z  RotationStandardAxis=+Z  RotationAngle=0.0  RotationAngleUnits=deg  RotationArbitraryAxis=[0 0 1]  RotationSequenceAxes=FollowerAxes  RotationSequence=XYX  RotationSequenceAngles=[0 0 0]  RotationSequenceAnglesUnits=deg  RotationMatrix=[1 0 0; 0 1 0; 0 0 1]  Quaternion=[1 0 0 0]  TranslationMethod=Cartesian  TranslationCartesianOffset=[wheelRadius/2 0 0]  TranslationCartesianOffsetUnits=m  TranslationStandardAxis=+Z  TranslationStandardOffset=0  TranslationStandardOffsetUnits=m  TranslationROffset=0  TranslationROffsetUnits=m  TranslationThetaOffset=0  TranslationThetaOffsetUnits=deg  TranslationZOffset=0  TranslationZOffsetUnits=m
  Rigid Transform4 : sm_lib/Frames and Transforms/Rigid Transform  RotationMethod=StandardAxis  FollAlignAxisA=+X  BaseAlignAxisA=+Y  FollAlignAxisB=+Y  BaseAlignAxisB=+Z  RotationStandardAxis=+Z  RotationAngle=180*choice  RotationAngleUnits=deg  RotationArbitraryAxis=[0 0 1]  RotationSequenceAxes=FollowerAxes  RotationSequence=XYX  RotationSequenceAngles=[0 0 0]  RotationSequenceAnglesUnits=deg  RotationMatrix=[1 0 0; 0 1 0; 0 0 1]  Quaternion=[1 0 0 0]  TranslationMethod=None  TranslationCartesianOffset=[0 0 0]  TranslationCartesianOffsetUnits=m  TranslationStandardAxis=+Z  TranslationStandardOffset=0  TranslationStandardOffsetUnits=m  TranslationROffset=0  TranslationROffsetUnits=m  TranslationThetaOffset=0  TranslationThetaOffsetUnits=deg  TranslationZOffset=0  TranslationZOffsetUnits=m
  Rigid Transform5 : sm_lib/Frames and Transforms/Rigid Transform  RotationMethod=None  FollAlignAxisA=+X  BaseAlignAxisA=+Y  FollAlignAxisB=+Y  BaseAlignAxisB=+Z  RotationStandardAxis=+Z  RotationAngle=0.0  RotationAngleUnits=deg  RotationArbitraryAxis=[0 0 1]  RotationSequenceAxes=FollowerAxes  RotationSequence=XYX  RotationSequenceAngles=[0 0 0]  RotationSequenceAnglesUnits=deg  RotationMatrix=[1 0 0; 0 1 0; 0 0 1]  Quaternion=[1 0 0 0]  TranslationMethod=Cartesian  TranslationCartesianOffset=[wheelRadius/2 0 0]  TranslationCartesianOffsetUnits=m  TranslationStandardAxis=+Z  TranslationStandardOffset=0  TranslationStandardOffsetUnits=m  TranslationROffset=0  TranslationROffsetUnits=m  TranslationThetaOffset=0  TranslationThetaOffsetUnits=deg  TranslationZOffset=0  TranslationZOffsetUnits=m
  Sensor Visuals : Subsystem
  Simscape Bus : SimscapeBus  HierarchyStrings=PlowSurface;RobotSurface;FloorSurface;Ref
  Simulink-PS Converter : nesl_utility/Simulink-PS Converter  PhysicalDomain=network_engine_domain  SubClassName=ps_input  LeftPortType=input  RightPortType=output  PseudoPeriodic=off  Frequencies=[]  NoiseDistribution=none  NoiseParameters=[]  Unit=1  AffineConversion=off  FilteringAndDerivatives=provide  SimscapeFilterOrder=1  InputFilterTimeConstant=0.05  UdotUserProvided=0
  Simulink-PS Converter1 : nesl_utility/Simulink-PS Converter  PhysicalDomain=network_engine_domain  SubClassName=ps_input  LeftPortType=input  RightPortType=output  PseudoPeriodic=off  Frequencies=[]  NoiseDistribution=none  NoiseParameters=[]  Unit=1  AffineConversion=off  FilteringAndDerivatives=provide  SimscapeFilterOrder=1  InputFilterTimeConstant=0.05  UdotUserProvided=0
  Solid : sm_lib/Body Elements/Brick Solid  BrickDimensions=[wheelRadius*0.8 wheelThickness*1.05 wheelThickness*1.05]  BrickDimensionsUnits=m  ExportEntireGeometry=off  InertiaType=CalculateFromGeometry  BasedOnType=Density  Density=1000  DensityUnits=kg/m^3  Mass=1  MassUnits=kg  CenterOfMass=[0 0 0]  CenterOfMassUnits=m  MomentsOfInertia=[1 1 1]  MomentsOfInertiaUnits=kg*m^2  ProductsOfInertia=[1 1 1]  ProductsOfInertiaUnits=kg*m^2  GraphicType=FromGeometry  MarkerShape=Sphere  MarkerSize=10  GraphicVisPropType=SimpleVisualProperties  GraphicDiffuseColor=[0.0 0.8 0.8]  GraphicOpacity=1.0  GraphicSpecularColor=[0.5 0.5 0.5 1.0]  GraphicAmbientColor=[0.15 0.15 0.15 1.0]  GraphicEmissiveColor=[0.0 0.0 0.0 1.0]  GraphicShininess=75  DoExposeReferenceFrame=on  SerializedFrames=<Frames/>
  Solid1 : sm_lib/Body Elements/Brick Solid  BrickDimensions=[wheelRadius*0.8 wheelThickness*1.05 wheelThickness*1.05]  BrickDimensionsUnits=m  ExportEntireGeometry=off  InertiaType=CalculateFromGeometry  BasedOnType=Density  Density=1000  DensityUnits=kg/m^3  Mass=1  MassUnits=kg  CenterOfMass=[0 0 0]  CenterOfMassUnits=m  MomentsOfInertia=[1 1 1]  MomentsOfInertiaUnits=kg*m^2  ProductsOfInertia=[1 1 1]  ProductsOfInertiaUnits=kg*m^2  GraphicType=FromGeometry  MarkerShape=Sphere  MarkerSize=10  GraphicVisPropType=SimpleVisualProperties  GraphicDiffuseColor=[0.0 0.8 0.8]  GraphicOpacity=1.0  GraphicSpecularColor=[0.5 0.5 0.5 1.0]  GraphicAmbientColor=[0.15 0.15 0.15 1.0]  GraphicEmissiveColor=[0.0 0.0 0.0 1.0]  GraphicShininess=75  DoExposeReferenceFrame=on  SerializedFrames=<Frames/>
  Spatial Contact Force : sm_lib/Forces and Torques/Spatial Contact Force  SenseSeparationDistance=off  NormalForceType=SmoothSpringDamper  NormalStiffness=1e4  NormalStiffnessUnits=N/m  NormalDamping=1e2  NormalDampingUnits=N/(m/s)  NormalTransitionRegionWidth=1e-2  NormalTransitionRegionWidthUnits=m  FrictionType=SmoothStickSlip  CoefficientOfStaticFriction=0.7  CoefficientOfDynamicFriction=0.5  FrictionalCriticalVelocity=1e-3  FrictionalCriticalVelocityUnits=m/s  SenseContactSignal=off  SensePenetrationDepth=off  SenseNormalVelocity=off  SenseTangentialVelocity=off  SensingForceTorqueDirection=BaseOnFollower  SensingForceTorqueResolutionFrame=ContactFrame  SenseNormalForce=off  SenseNormalForceMagnitude=off  SenseNormalTorque=off  SenseFrictionalForce=off  SenseFrictionalForceMagnitude=off  SenseFrictionalTorque=off  SenseTotalForce=off  SenseTotalTorque=off  SenseContactBaseRotation=off  SenseContactBaseTranslation=off  SenseContactFollowerRotation=off  SenseContactFollowerTranslation=off  ZeroCrossDetectContactStartAndEnd=off
  Spatial Contact Force1 : sm_lib/Forces and Torques/Spatial Contact Force  SenseSeparationDistance=off  NormalForceType=SmoothSpringDamper  NormalStiffness=1e4  NormalStiffnessUnits=N/m  NormalDamping=1e2  NormalDampingUnits=N/(m/s)  NormalTransitionRegionWidth=1e-2  NormalTransitionRegionWidthUnits=m  FrictionType=SmoothStickSlip  CoefficientOfStaticFriction=0.7  CoefficientOfDynamicFriction=0.5  FrictionalCriticalVelocity=1e-3  FrictionalCriticalVelocityUnits=m/s  SenseContactSignal=off  SensePenetrationDepth=off  SenseNormalVelocity=off  SenseTangentialVelocity=off  SensingForceTorqueDirection=BaseOnFollower  SensingForceTorqueResolutionFrame=ContactFrame  SenseNormalForce=off  SenseNormalForceMagnitude=off  SenseNormalTorque=off  SenseFrictionalForce=off  SenseFrictionalForceMagnitude=off  SenseFrictionalTorque=off  SenseTotalForce=off  SenseTotalTorque=off  SenseContactBaseRotation=off  SenseContactBaseTranslation=off  SenseContactFollowerRotation=off  SenseContactFollowerTranslation=off  ZeroCrossDetectContactStartAndEnd=off
  Transform Sensor1 : sm_lib/Frames and Transforms/Transform Sensor  MeasurementFrame=World  RotationSequence=XYX  SenseAngle=on  SenseAxis=off  SenseQ=off  SenseR=off  SenseRotationSequence=off  SenseOmegaX=off  SenseOmegaY=off  SenseOmegaZ=off  SenseOmega=off  SenseQDot=off  SenseRDot=off  SenseRotationSequenceDot=off  SenseAlphaX=off  SenseAlphaY=off  SenseAlphaZ=off  SenseAlpha=off  SenseQDDot=off  SenseRDDot=off  SenseX=off  SenseY=off  SenseZ=off  SenseXYZ=off  SenseRad=off  SenseAzim=off  SenseDist=off  SenseInc=off  SenseXDot=off  SenseYDot=off  SenseZDot=off  SenseXYZDot=off  SenseRadDot=off  SenseAzimDot=off  SenseDistDot=off  SenseIncDot=off  SenseXDDot=off  SenseYDDot=off  SenseZDDot=off  SenseXYZDDot=off  SenseRadDDot=off  SenseAzimDDot=off  SenseDistDDot=off  SenseIncDDot=off
  Robot : PMIOPort  Side=Right
  tag scope: R1motor1q=global, R1motor1w=global, R1motor2q=global, R1motor2w=global, R1tAngle=global, R1tPose=global, R1tRate=global, R1xPose=global, R1yPose=global
  wires:
  PS-Simulink Converter8/1 -> [R1tAngle]
  PS-Simulink Converter7/1 -> [R1tRate]
  [R1motor2t] -> Filter1/1
  [R1motor1t] -> Filter/1(y)
  Gain1/1 -> Simulink-PS Converter1/1
  Gain/1 -> Simulink-PS Converter/1
  Filter/1(x) -> Gain/1
  Filter1/1 -> Gain1/1
  PS-Simulink Converter4/1 -> Interpreted MATLAB Function2/1
  PS-Simulink Converter3/1 -> Interpreted MATLAB Function1/1
  PS-Simulink Converter2/1 -> [R1tPose]  "thetaPose"
  Interpreted MATLAB Function1/1 -> [R1xPose]  "xPose"
  Interpreted MATLAB Function2/1 -> [R1yPose]  "yPose"
  PS-Simulink Converter1/1 -> [R1motor2w]  "motor2w"
  PS-Simulink Converter/1 -> [R1motor2q]  "motor2q"
  PS-Simulink Converter5/1 -> [R1motor1q]  "motor1pose"
  PS-Simulink Converter6/1 -> [R1motor1w]  "motor1w"
  connections:
  Body/RConn1 -- Simscape Bus/LConn2
  Plow/RConn1 -- Simscape Bus/LConn1
  Spatial Contact Force/LConn1 -- Spatial Contact Force1/LConn1 -- Simscape Bus/LConn3
  Spatial Contact Force1/RConn1 -- Right Wheel/LConn1
  Spatial Contact Force/RConn1 -- Left Wheel/LConn1
  Rigid Transform5/RConn1 -- Solid1/RConn1
  Rigid Transform3/RConn1 -- Solid/RConn1
  Robot/RConn1 -- Simscape Bus/RConn1
  Transform Sensor1/RConn2 -- PS-Simulink Converter8/LConn1
  Planar Joint2/RConn5 -- PS-Simulink Converter7/LConn1
  Prismatic Joint/RConn1 -- Rigid Transform2/LConn1
  Rigid Transform4/LConn1 -- Transform Sensor1/RConn1 -- Planar Joint2/RConn1
  Rigid Transform4/RConn1 -- Body/LConn1 -- Plow/LConn1 -- Rigid Transform1/LConn1 -- Rigid Transform/LConn1 -- Sensor Visuals/LConn1
  Motor1/RConn1 -- Left Wheel/RConn1 -- Rigid Transform5/LConn1
  Motor2/LConn1 -- Rigid Transform1/RConn1
  Prismatic Joint/LConn1 -- Transform Sensor1/LConn1 -- Simscape Bus/LConn4
  Planar Joint2/LConn1 -- Rigid Transform2/RConn1
  Motor1/LConn1 -- Rigid Transform/RConn1
  Motor2/RConn1 -- Rigid Transform3/LConn1 -- Right Wheel/RConn1
  Simulink-PS Converter1/RConn1 -- Motor2/LConn2
  Simulink-PS Converter/RConn1 -- Motor1/LConn2
  Planar Joint2/RConn2 -- PS-Simulink Converter3/LConn1
  Planar Joint2/RConn3 -- PS-Simulink Converter4/LConn1
  Planar Joint2/RConn4 -- PS-Simulink Converter2/LConn1
  Motor1/RConn2 -- PS-Simulink Converter5/LConn1
  Motor1/RConn3 -- PS-Simulink Converter6/LConn1
  PS-Simulink Converter/LConn1 -- Motor2/RConn2
  PS-Simulink Converter1/LConn1 -- Motor2/RConn3

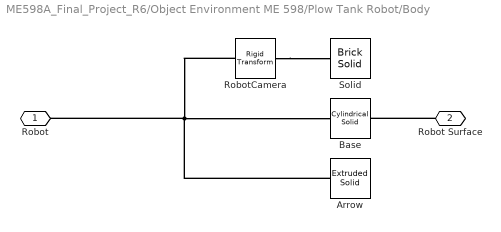
== system ME598A_Final_Project_R6/Object Environment ME 598/Plow Tank Robot/Body ==
  Arrow : sm_lib/Body Elements/Extruded Solid  ExtrusionType=Regular  PolygonNumSides=3  PolygonOuterRadius=wheelBase/2-wheelBase*0.15  PolygonOuterRadiusUnits=m  ExportEntireGeometry=off  ExtrusionCrossSection=[1 1; -1 1; -1 -1; 1 -1]  ExtrusionCrossSectionUnits=m  ExportConvexHullGeometry=off  ExtrusionLength=1.3*chassisThickness  ExtrusionLengthUnits=m  InertiaType=PointMass  BasedOnType=Density  Density=1000  DensityUnits=kg/m^3  Mass=0.2  MassUnits=kg  CenterOfMass=[0 0 0]  CenterOfMassUnits=m  MomentsOfInertia=[1 1 1]  MomentsOfInertiaUnits=kg*m^2  ProductsOfInertia=[1 1 1]  ProductsOfInertiaUnits=kg*m^2  GraphicType=FromGeometry  MarkerShape=Sphere  MarkerSize=10  GraphicVisPropType=SimpleVisualProperties  GraphicDiffuseColor=[0.8 0.0 1.0]  GraphicOpacity=1.0  GraphicSpecularColor=[0.5 0.5 0.5 1.0]  GraphicAmbientColor=[0.15 0.15 0.15 1.0]  GraphicEmissiveColor=[0.0 0.0 0.0 1.0]  GraphicShininess=75  DoExposeReferenceFrame=on  SerializedFrames=<Frames/>
  Base : sm_lib/Body Elements/Cylindrical Solid  CylinderRadius=(wheelBase-wheelThickness)/2  CylinderRadiusUnits=m  CylinderLength=chassisThickness  CylinderLengthUnits=m  ExportEntireGeometry=on  InertiaType=CalculateFromGeometry  BasedOnType=Mass  Density=chassisMass  DensityUnits=kg/m^3  Mass=chassisMass  MassUnits=kg  CenterOfMass=[0 0 0]  CenterOfMassUnits=m  MomentsOfInertia=[1 1 1]  MomentsOfInertiaUnits=kg*m^2  ProductsOfInertia=[1 1 1]  ProductsOfInertiaUnits=kg*m^2  GraphicType=FromGeometry  MarkerShape=Sphere  MarkerSize=10  GraphicVisPropType=SimpleVisualProperties  GraphicDiffuseColor=chassisColor  GraphicOpacity=1.0  GraphicSpecularColor=[0.5 0.5 0.5 1.0]  GraphicAmbientColor=[0.15 0.15 0.15 1.0]  GraphicEmissiveColor=[0.0 0.0 0.0 1.0]  GraphicShininess=75  DoExposeReferenceFrame=on  SerializedFrames=<Frames/>
  RobotCamera : sm_lib/Frames and Transforms/Rigid Transform  RotationMethod=StandardAxis  FollAlignAxisA=+X  BaseAlignAxisA=+Y  FollAlignAxisB=+Y  BaseAlignAxisB=+Z  RotationStandardAxis=+Y  RotationAngle=20  RotationAngleUnits=deg  RotationArbitraryAxis=[0 0 1]  RotationSequenceAxes=FollowerAxes  RotationSequence=XYX  RotationSequenceAngles=[0 0 0]  RotationSequenceAnglesUnits=deg  RotationMatrix=[1 0 0; 0 1 0; 0 0 1]  Quaternion=[1 0 0 0]  TranslationMethod=Cartesian  TranslationCartesianOffset=[-0.5 0 0.35]  TranslationCartesianOffsetUnits=m  TranslationStandardAxis=+Z  TranslationStandardOffset=0  TranslationStandardOffsetUnits=m  TranslationROffset=0  TranslationROffsetUnits=m  TranslationThetaOffset=0  TranslationThetaOffsetUnits=deg  TranslationZOffset=0  TranslationZOffsetUnits=m
  Solid : sm_lib/Body Elements/Brick Solid  BrickDimensions=[0.001 0.001 0.001]  BrickDimensionsUnits=m  ExportEntireGeometry=off  InertiaType=PointMass  BasedOnType=Density  Density=1000  DensityUnits=kg/m^3  Mass=0.00001  MassUnits=kg  CenterOfMass=[0 0 0]  CenterOfMassUnits=m  MomentsOfInertia=[1 1 1]  MomentsOfInertiaUnits=kg*m^2  ProductsOfInertia=[1 1 1]  ProductsOfInertiaUnits=kg*m^2  GraphicType=FromGeometry  MarkerShape=Sphere  MarkerSize=10  GraphicVisPropType=SimpleVisualProperties  GraphicDiffuseColor=[0.5 0.5 0.5]  GraphicOpacity=0  GraphicSpecularColor=[0.5 0.5 0.5 1.0]  GraphicAmbientColor=[0.15 0.15 0.15 1.0]  GraphicEmissiveColor=[0.0 0.0 0.0 1.0]  GraphicShininess=75  DoExposeReferenceFrame=on  SerializedFrames=<Frames/>
  Robot : PMIOPort  Side=Left
  Robot Surface : PMIOPort  Port=2  Side=Right
  connections:
  Robot Surface/RConn1 -- Base/LConn1
  RobotCamera/RConn1 -- Solid/RConn1
  Arrow/RConn1 -- Robot/RConn1 -- RobotCamera/LConn1 -- Base/RConn1

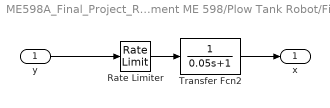
== system ME598A_Final_Project_R6/Object Environment ME 598/Plow Tank Robot/Filter ==
  y : Inport
  Rate Limiter : RateLimiter  RisingSlewLimit=300  FallingSlewLimit=-300  SampleTimeMode=inherited
  Transfer Fcn2 : TransferFcn  Denominator=[0.05 1]
  x : Outport  VectorParamsAs1DForOutWhenUnconnected=off
  wires:
  Rate Limiter/1 -> Transfer Fcn2/1
  Transfer Fcn2/1 -> x/1
  y/1 -> Rate Limiter/1

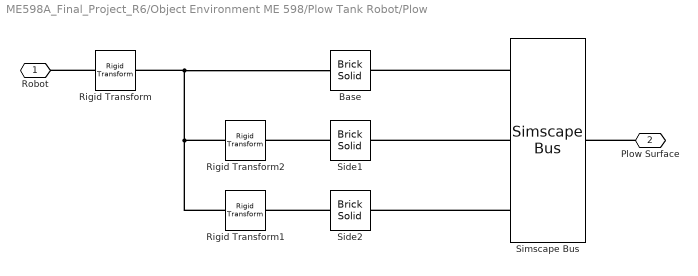
== system ME598A_Final_Project_R6/Object Environment ME 598/Plow Tank Robot/Plow ==
  Base : sm_lib/Body Elements/Brick Solid  BrickDimensions=[0.02 wheelBase wheelRadius]  BrickDimensionsUnits=m  ExportEntireGeometry=on  InertiaType=CalculateFromGeometry  BasedOnType=Mass  Density=chassisMass  DensityUnits=kg/m^3  Mass=chassisMass  MassUnits=kg  CenterOfMass=[0 0 0]  CenterOfMassUnits=m  MomentsOfInertia=[1 1 1]  MomentsOfInertiaUnits=kg*m^2  ProductsOfInertia=[1 1 1]  ProductsOfInertiaUnits=kg*m^2  GraphicType=FromGeometry  MarkerShape=Sphere  MarkerSize=10  GraphicVisPropType=SimpleVisualProperties  GraphicDiffuseColor=[0.2 0.8 0.0]  GraphicOpacity=1.0  GraphicSpecularColor=[0.5 0.5 0.5 1.0]  GraphicAmbientColor=[0.15 0.15 0.15 1.0]  GraphicEmissiveColor=[0.0 0.0 0.0 1.0]  GraphicShininess=75  DoExposeReferenceFrame=on  SerializedFrames=<Frames/>
  Rigid Transform : sm_lib/Frames and Transforms/Rigid Transform  RotationMethod=None  FollAlignAxisA=+X  BaseAlignAxisA=+Y  FollAlignAxisB=+Y  BaseAlignAxisB=+Z  RotationStandardAxis=+Z  RotationAngle=0.0  RotationAngleUnits=deg  RotationArbitraryAxis=[0 0 1]  RotationSequenceAxes=FollowerAxes  RotationSequence=XYX  RotationSequenceAngles=[0 0 0]  RotationSequenceAnglesUnits=deg  RotationMatrix=[1 0 0; 0 1 0; 0 0 1]  Quaternion=[1 0 0 0]  TranslationMethod=Cartesian  TranslationCartesianOffset=[wheelBase/2-0.02 0 0]  TranslationCartesianOffsetUnits=m  TranslationStandardAxis=+Z  TranslationStandardOffset=0  TranslationStandardOffsetUnits=m  TranslationROffset=0  TranslationROffsetUnits=m  TranslationThetaOffset=0  TranslationThetaOffsetUnits=deg  TranslationZOffset=0  TranslationZOffsetUnits=m
  Rigid Transform1 : sm_lib/Frames and Transforms/Rigid Transform  RotationMethod=None  FollAlignAxisA=+X  BaseAlignAxisA=+Y  FollAlignAxisB=+Y  BaseAlignAxisB=+Z  RotationStandardAxis=+Z  RotationAngle=0.0  RotationAngleUnits=deg  RotationArbitraryAxis=[0 0 1]  RotationSequenceAxes=FollowerAxes  RotationSequence=XYX  RotationSequenceAngles=[0 0 0]  RotationSequenceAnglesUnits=deg  RotationMatrix=[1 0 0; 0 1 0; 0 0 1]  Quaternion=[1 0 0 0]  TranslationMethod=Cartesian  TranslationCartesianOffset=[0.09 wheelBase/2 0]  TranslationCartesianOffsetUnits=m  TranslationStandardAxis=+Z  TranslationStandardOffset=0  TranslationStandardOffsetUnits=m  TranslationROffset=0  TranslationROffsetUnits=m  TranslationThetaOffset=0  TranslationThetaOffsetUnits=deg  TranslationZOffset=0  TranslationZOffsetUnits=m
  Rigid Transform2 : sm_lib/Frames and Transforms/Rigid Transform  RotationMethod=None  FollAlignAxisA=+X  BaseAlignAxisA=+Y  FollAlignAxisB=+Y  BaseAlignAxisB=+Z  RotationStandardAxis=+Z  RotationAngle=0.0  RotationAngleUnits=deg  RotationArbitraryAxis=[0 0 1]  RotationSequenceAxes=FollowerAxes  RotationSequence=XYX  RotationSequenceAngles=[0 0 0]  RotationSequenceAnglesUnits=deg  RotationMatrix=[1 0 0; 0 1 0; 0 0 1]  Quaternion=[1 0 0 0]  TranslationMethod=Cartesian  TranslationCartesianOffset=[0.09 -wheelBase/2 0]  TranslationCartesianOffsetUnits=m  TranslationStandardAxis=+Z  TranslationStandardOffset=0  TranslationStandardOffsetUnits=m  TranslationROffset=0  TranslationROffsetUnits=m  TranslationThetaOffset=0  TranslationThetaOffsetUnits=deg  TranslationZOffset=0  TranslationZOffsetUnits=m
  Side1 : sm_lib/Body Elements/Brick Solid  BrickDimensions=[0.2 0.02 wheelRadius]  BrickDimensionsUnits=m  ExportEntireGeometry=on  InertiaType=CalculateFromGeometry  BasedOnType=Mass  Density=chassisMass  DensityUnits=kg/m^3  Mass=chassisMass  MassUnits=kg  CenterOfMass=[0 0 0]  CenterOfMassUnits=m  MomentsOfInertia=[1 1 1]  MomentsOfInertiaUnits=kg*m^2  ProductsOfInertia=[1 1 1]  ProductsOfInertiaUnits=kg*m^2  GraphicType=FromGeometry  MarkerShape=Sphere  MarkerSize=10  GraphicVisPropType=SimpleVisualProperties  GraphicDiffuseColor=[0.2 0.8 0.0]  GraphicOpacity=1.0  GraphicSpecularColor=[0.5 0.5 0.5 1.0]  GraphicAmbientColor=[0.15 0.15 0.15 1.0]  GraphicEmissiveColor=[0.0 0.0 0.0 1.0]  GraphicShininess=75  DoExposeReferenceFrame=on  SerializedFrames=<Frames/>
  Side2 : sm_lib/Body Elements/Brick Solid  BrickDimensions=[0.2 0.02 wheelRadius]  BrickDimensionsUnits=m  ExportEntireGeometry=on  InertiaType=CalculateFromGeometry  BasedOnType=Mass  Density=chassisMass  DensityUnits=kg/m^3  Mass=chassisMass  MassUnits=kg  CenterOfMass=[0 0 0]  CenterOfMassUnits=m  MomentsOfInertia=[1 1 1]  MomentsOfInertiaUnits=kg*m^2  ProductsOfInertia=[1 1 1]  ProductsOfInertiaUnits=kg*m^2  GraphicType=FromGeometry  MarkerShape=Sphere  MarkerSize=10  GraphicVisPropType=SimpleVisualProperties  GraphicDiffuseColor=[0.2 0.8 0.0]  GraphicOpacity=1.0  GraphicSpecularColor=[0.5 0.5 0.5 1.0]  GraphicAmbientColor=[0.15 0.15 0.15 1.0]  GraphicEmissiveColor=[0.0 0.0 0.0 1.0]  GraphicShininess=75  DoExposeReferenceFrame=on  SerializedFrames=<Frames/>
  Simscape Bus : SimscapeBus  HierarchyStrings=Base;Side1;Side2
  Robot : PMIOPort  Side=Left
  Plow Surface : PMIOPort  Port=2  Side=Right
  connections:
  Plow Surface/RConn1 -- Simscape Bus/RConn1
  Simscape Bus/LConn3 -- Side2/LConn1
  Simscape Bus/LConn2 -- Side1/LConn1
  Simscape Bus/LConn1 -- Base/LConn1
  Rigid Transform2/LConn1 -- Rigid Transform1/LConn1 -- Base/RConn1 -- Rigid Transform/RConn1
  Rigid Transform/LConn1 -- Robot/RConn1
  Side2/RConn1 -- Rigid Transform1/RConn1
  Side1/RConn1 -- Rigid Transform2/RConn1

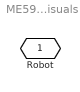
== system ME598A_Final_Project_R6/Object Environment ME 598/Plow Tank Robot/Sensor Visuals ==
  Robot : PMIOPort  Side=Left
